simulink model "aula_07"  (R2026a)
settings: Solver=VariableStepAuto  StopTime=tsim  MaxStep=1e-1
values from neighbouring files (symbols this model uses):
  ae0 = 0.6    [Lab11.m]    (also in Lab11_pronto.m; Lab_7.m; aula08.m; aula08_lab.m)
  as0 = 0.5    [Lab11.m]    (also in Lab11_pronto.m; Lab_7.m; aula08.m; aula08_lab.m)
  H0 = ((ke*ae0)/(ks*as0*sqrt(2*g)))^2    [Lab11.m]    (also in Lab11_pronto.m = ((ke*ae0)/(ks*as0*sqrt(2*gg)))^2; Lab_7.m; aula08.m; aula08_lab.m)
  hyst = 0.02    [Lab_7.m]
  tsim = 2500    [Lab11.m]    (also in Lab11_pronto.m; Lab_7.m = 500; aula08.m = 500; aula08_lab.m = 500)
libraries: cstblocks_lti x4
settings Model: Creator=Prof. Daniel Cruz

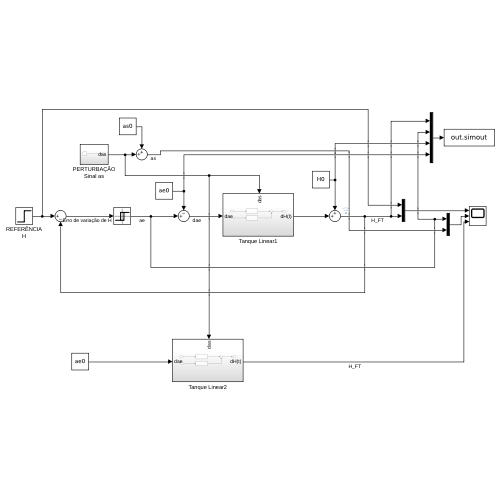
[thumbnail: Simulink's stored preview of the top-level diagram]
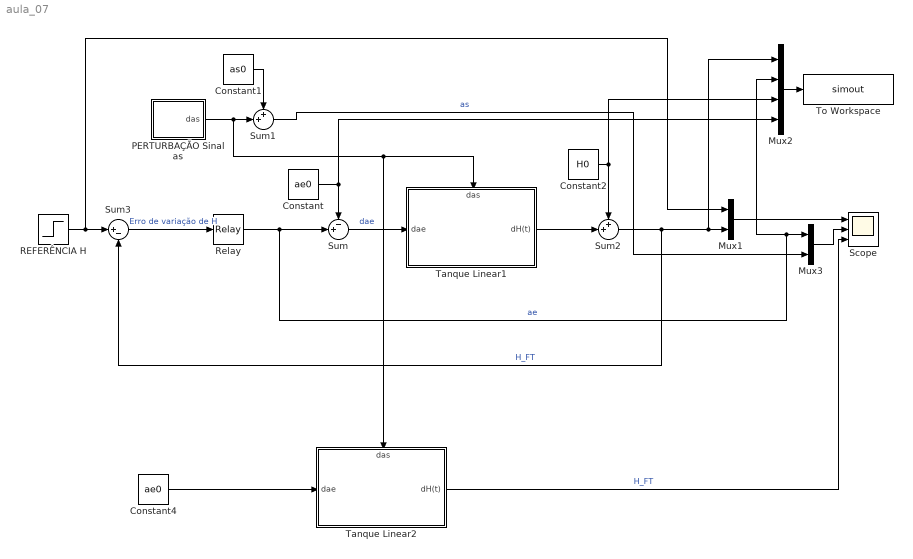
== system aula_07 ==
  Constant : Constant  Value=ae0
  Constant1 : Constant  Value=as0
  Constant2 : Constant  Value=H0
  Constant4 : Constant  Value=ae0
  Mux1 : Mux  Inputs=2
  Mux2 : Mux
  Mux3 : Mux  Inputs=2
  PERTURBAÇÃO Sinal as : Subsystem
  REFERÊNCIA H : Step  InitialValue=H0  FinalValue=H_ref  SampleTime=0
  Relay : Relay  OnSwitchValue=+hyst  OffSwitchValue=-hyst  OnOutputValue=ae_on  OffOutputValue=ae_off
  Scope : Scope  NumInputPorts=3
      settings: ActiveDisplayYMinimum=0.67139  ActiveDisplayYMaximum=1.03243
  Sum : Sum  Inputs=-+|
  Sum1 : Sum  Inputs=++|
  Sum2 : Sum  Inputs=++|
  Sum3 : Sum  Inputs=|+-
  Tanque Linear1 : Subsystem
      settings: PortSchema="{\"entries\":[{\"content\":{\"sides\":[{\"content\":{\"connectorIds\":[\"In1\"]},\"type\":\"ConnectorPlacement.EquallySpacedRectSide\",\"uuid\":\"f67b16a6-d13c-4ce1-92bf-a3b7b78f55b2\"},{\"content\":{\"connectorIds\":[\"Out1\"],\"side\":\"RIGHT\"},\"type\":\"ConnectorPlacement.EquallySpacedRectSide\",\"uuid\":\"6dfa0371-c497-4466-b77b-e5c5fe181385\"},{\"content\":{\"connectorIds\":[\"In2\"],\"side\":\"TOP\"},\"type\":\"ConnectorPlacement.EquallySpacedRectSide\",\"uuid\":\"6450f77e-1436-4798-86e5-b0a6495bdb9b\"}]},\"type\":\"ConnectorPlacement.EquallySpacedConnector\",\"uuid\":\"6402b57b-709e-4d3a-bcb1-330d3ba010a6\"}],\"packageUris\":[\"http://schema.mathworks.com/mf0/Connector/R2020b\"],\"version\":\"1.0\"}"
  Tanque Linear2 : Subsystem
      settings: PortSchema="{\"entries\":[{\"content\":{\"sides\":[{\"content\":{\"connectorIds\":[\"In1\"]},\"type\":\"ConnectorPlacement.EquallySpacedRectSide\",\"uuid\":\"f67b16a6-d13c-4ce1-92bf-a3b7b78f55b2\"},{\"content\":{\"connectorIds\":[\"Out1\"],\"side\":\"RIGHT\"},\"type\":\"ConnectorPlacement.EquallySpacedRectSide\",\"uuid\":\"6dfa0371-c497-4466-b77b-e5c5fe181385\"},{\"content\":{\"connectorIds\":[\"In2\"],\"side\":\"TOP\"},\"type\":\"ConnectorPlacement.EquallySpacedRectSide\",\"uuid\":\"6450f77e-1436-4798-86e5-b0a6495bdb9b\"}]},\"type\":\"ConnectorPlacement.EquallySpacedConnector\",\"uuid\":\"6402b57b-709e-4d3a-bcb1-330d3ba010a6\"}],\"packageUris\":[\"http://schema.mathworks.com/mf0/Connector/R2020b\"],\"version\":\"1.0\"}"
  To Workspace : ToWorkspace  VariableName=simout  SaveFormat=Timeseries  SampleTime=-1
  wires:
  Constant/1 -> Mux2/4, Sum/1
  Constant1/1 -> Sum1/1
  PERTURBAÇÃO Sinal as/1(das) -> Tanque Linear2/2(das), Tanque Linear1/2(das), Sum1/2
  Tanque Linear1/1(dH(t)) -> Sum2/2
  Constant2/1 -> Sum2/1, Mux2/3
  Sum2/1 -> Sum3/2, Mux2/1, Mux1/2  "H_FT"
  Mux1/1 -> Scope/1
  Sum1/1 -> Mux3/2  "as"
  REFERÊNCIA H/1 -> Mux1/1, Sum3/1
  Sum3/1 -> Relay/1  "Erro de variação de H"
  Relay/1 -> Mux3/1, Mux2/2, Sum/2  "ae"
  Sum/1 -> Tanque Linear1/1(dae)  "dae"
  Mux2/1 -> To Workspace/1
  Mux3/1 -> Scope/2
  Tanque Linear2/1(dH(t)) -> Scope/3  "H_FT"
  Constant4/1 -> Tanque Linear2/1(dae)

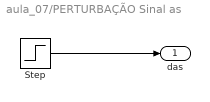
== system aula_07/PERTURBAÇÃO Sinal as ==
  Step : Step  Time=(2/5)*tsim  FinalValue=0.05  SampleTime=0
  das : Outport
  wires:
  Step/1 -> das/1

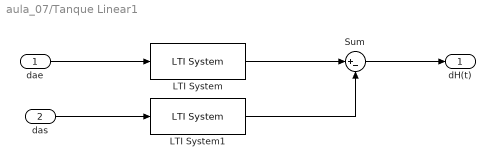
== system aula_07/Tanque Linear1 ==
  dae : Inport
  das : Inport  Port=2
  LTI System : cstblocks_lti/LTI System  sys=G  IC=[]  PadeOrder=0
  LTI System1 : cstblocks_lti/LTI System  sys=G_as  IC=[]  PadeOrder=0
  Sum : Sum  Inputs=|+-
  dH(t) : Outport
  wires:
  dae/1 -> LTI System/1
  das/1 -> LTI System1/1
  LTI System/1 -> Sum/1
  LTI System1/1 -> Sum/2
  Sum/1 -> dH(t)/1

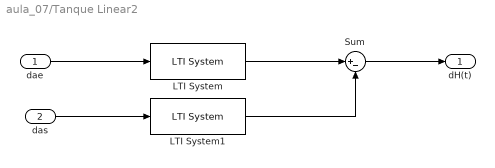
== system aula_07/Tanque Linear2 ==
  dae : Inport
  das : Inport  Port=2
  LTI System : cstblocks_lti/LTI System  sys=G  IC=[]  PadeOrder=0
  LTI System1 : cstblocks_lti/LTI System  sys=G_as  IC=[]  PadeOrder=0
  Sum : Sum  Inputs=|+-
  dH(t) : Outport
  wires:
  dae/1 -> LTI System/1
  das/1 -> LTI System1/1
  LTI System/1 -> Sum/1
  LTI System1/1 -> Sum/2
  Sum/1 -> dH(t)/1
